simulink subsystem "load_current"  (R2025b)
settings: Solver=VariableStepAuto  StartTime=0.0  StopTime=10.0  RelTol=1e-3
settings Model: Creator=lenovo  LastModifiedBy=lenovo

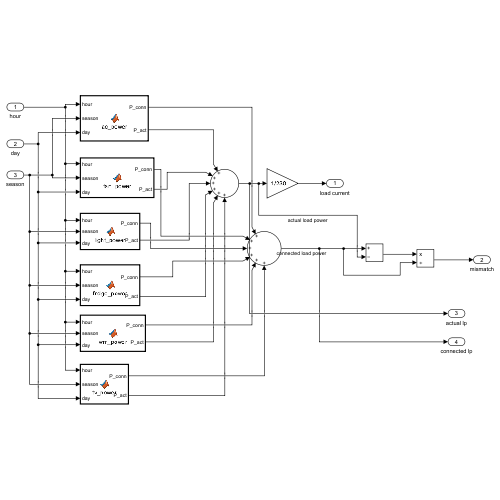
[thumbnail: Simulink's stored preview of the top-level diagram]
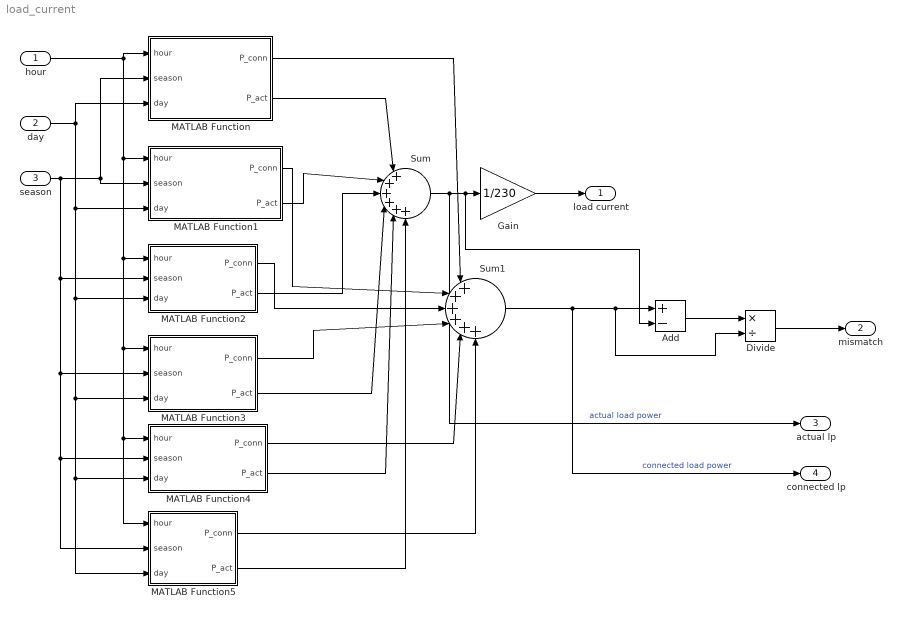
== system load_current ==
  hour : Inport
  day : Inport  Port=2
  season : Inport  Port=3
  Add : Sum  Inputs=+-
  Divide : Product  Inputs=*/
  Gain : Gain  Gain=1/230
  MATLAB Function : MATLAB Function  TreatAsAtomicUnit=on
  MATLAB Function1 : MATLAB Function  TreatAsAtomicUnit=on
  MATLAB Function2 : MATLAB Function  TreatAsAtomicUnit=on
  MATLAB Function3 : MATLAB Function  TreatAsAtomicUnit=on
  MATLAB Function4 : MATLAB Function  TreatAsAtomicUnit=on
  MATLAB Function5 : MATLAB Function  TreatAsAtomicUnit=on
  Sum : Sum  Inputs=|++++++
  Sum1 : Sum  Inputs=|++++++
  load current : Outport
  mismatch : Outport  Port=2
  actual lp : Outport  Port=3
  connected lp : Outport  Port=4
  wires:
  hour/1 -> MATLAB Function5/1(hour), MATLAB Function4/1(hour), MATLAB Function3/1(hour), MATLAB Function2/1(hour), MATLAB Function1/1(hour), MATLAB Function/1(hour)
  season/1 -> MATLAB Function5/2(season), MATLAB Function4/2(season), MATLAB Function3/2(season), MATLAB Function2/2(season), MATLAB Function1/2(season), MATLAB Function/2(season)
  day/1 -> MATLAB Function5/3(day), MATLAB Function4/3(day), MATLAB Function3/3(day), MATLAB Function2/3(day), MATLAB Function1/3(day), MATLAB Function/3(day)
  Sum/1 -> actual lp/1, Add/2, Gain/1  "actual load power"
  Gain/1 -> load current/1
  MATLAB Function/2(P_act) -> Sum/1
  MATLAB Function1/2(P_act) -> Sum/2
  MATLAB Function2/2(P_act) -> Sum/3
  MATLAB Function3/2(P_act) -> Sum/4
  MATLAB Function4/2(P_act) -> Sum/5
  MATLAB Function5/2(P_act) -> Sum/6
  MATLAB Function/1(P_conn) -> Sum1/1
  MATLAB Function1/1(P_conn) -> Sum1/2
  MATLAB Function2/1(P_conn) -> Sum1/3
  MATLAB Function3/1(P_conn) -> Sum1/4
  MATLAB Function4/1(P_conn) -> Sum1/5
  MATLAB Function5/1(P_conn) -> Sum1/6
  Sum1/1 -> connected lp/1, Divide/2, Add/1  "connected load power"
  Add/1 -> Divide/1
  Divide/1 -> mismatch/1

== matlab function load_current/MATLAB Function ==
  settings: updateMethod=DISCRETE
  data: hour input; P_conn output; season input; day input; P_act output
function [P_conn, P_act] = ac_power(hour, season, day)


if hour >= 12 && hour <= 18
    base = 1500;
elseif hour >= 20 && hour <= 23
    base = 1200;
else
    base = 200;
end

% Seasonal effect
if season == 1       % Summer
    scale = 1.4;
elseif season == 2   % Rainy
    scale = 1.0;
else                % Winter
    scale = 0.5;
end

P_conn = base * scale;
if rand < 0.9
    P_act = P_conn;
else
    P_act = P_conn * (0.9 + 0.2*rand);
end
isWeekend = (mod(day,7)==6)||(mod(day,7)==0);
% Weekend (slightly higher usage)
if isWeekend && rand < 0.3
    P_act = P_act * 1.05;
end

if rand < 0.02
    P_act = 0;
end

% Rare spike
if rand < 0.01
    P_act = P_act * 1.3;
end

% Small noise
P_act = P_act + 0.02 * P_conn * randn;

end

== matlab function load_current/MATLAB Function1 ==
  settings: updateMethod=DISCRETE
  data: hour input; P_conn output; season input; day input; P_act output
function [P_conn, P_act] = ac_power(hour, season, day)

% --- CONNECTED LOAD ---
if hour >= 12 && hour <= 18
    base = 1500;
elseif hour >= 20 && hour <= 23
    base = 1200;
else
    base = 200;
end

% Seasonal effect
if season == 1       % Summer
    scale = 1.4;
elseif season == 2   % Rainy
    scale = 1.0;
else                % Winter
    scale = 0.5;
end

P_conn = base * scale;

% --- ACTUAL LOAD ---
if rand < 0.9
    P_act = P_conn;
else
    P_act = P_conn * (0.9 + 0.2*rand);
end
isWeekend = (mod(day,7)==6)||(mod(day,7)==0);
% Weekend (slightly higher usage)
if isWeekend && rand < 0.3
    P_act = P_act * 1.05;
end

% Rare OFF
if rand < 0.02
    P_act = 0;
end

% Rare spike
if rand < 0.01
    P_act = P_act * 1.3;
end

% Small noise
P_act = P_act + 0.02 * P_conn * randn;

end

== matlab function load_current/MATLAB Function2 ==
  data: hour input; season input; P_conn output; day input; P_act output
function [P_conn, P_act] = light_power(hour, season, day)

if hour >= 18 || hour <= 6
    base = 100;
else
    base = 20;
end

P_conn = base;

if rand < 0.9
    P_act = P_conn;
else
    P_act = P_conn * (0.9 + 0.2*rand);
end
isWeekend = (mod(day,7)==6)||(mod(day,7)==0);
% Weekend (more usage)
if isWeekend && rand < 0.4
    P_act = P_act * 1.1;
end

% Rare OFF
if rand < 0.02
    P_act = 0;
end

% Noise
P_act = P_act + 0.02 * P_conn * randn;

end

== matlab function load_current/MATLAB Function3 ==
  data: hour input; season input; P_conn output; day input; P_act output
function [P_conn, P_act] = fridge_power(hour, season, day)

P_conn = 150;

% Mostly constant
if rand < 0.9
    P_act = P_conn;
else
    P_act = 150 + 30*sin(2*pi*hour/2);
end

% Seasonal slight variation
if season == 1
    P_act = P_act * 1.05;
end

% Noise
P_act = P_act + 5*randn;

end

== matlab function load_current/MATLAB Function4 ==
  data: hour input; season input; P_conn output; day input; P_act output
function [P_conn, P_act] = wm_power(hour, season, day)

P_conn = 500;

isWeekend = (mod(day,7)==6)||(mod(day,7)==0);

% Usage probability
if isWeekend
    prob = 0.2;
else
    prob = 0.08;
end

if rand < prob && hour >= 8 && hour <= 20
    P_act = 500;
else
    P_act = 0;
end

end

== matlab function load_current/MATLAB Function5 ==
  data: hour input; season input; P_conn output; day input; P_act output
function [P_conn, P_act] = tv_power(hour, season, day)

if hour >= 18 && hour <= 23
    base = 120;
else
    base = 20;
end

P_conn = base;

if rand < 0.9
    P_act = P_conn;
else
    P_act = P_conn * (0.9 + 0.2*rand);
end
isWeekend = (mod(day,7)==6)||(mod(day,7)==0);
% Weekend binge
if isWeekend && rand < 0.5
    P_act = P_act * 1.1;
end

% Rare OFF
if rand < 0.03
    P_act = 0;
end

% Noise
P_act = P_act + 0.02 * P_conn * randn;

end
